simulink model "s_c107m32k_vlbi"  (R2018a)
settings: Solver=VariableStepDiscrete  StartTime=0.0  StopTime=(2^15)*10  RelTol=1e-3
undefined symbols (not defined in the file): fft_stages, n_bits_xengs
libraries: xbsIndex_r4 x23049, casper_library_misc x45, xps_library x4, casper_library_scopes x3, simulink x2
(part 96 of 201)

== system s_c107m32k_vlbi/cd_hmc/hmc_delay/ctrl_pol1 ==
  note: Stall the address increment by 1 cycle as two
      | 128bit words need to be concatenated into one 256bit word
  note: Add a 512 address offset. This is so that the read and write dont clash,
      | and to allow sufficicient time for the HMC to perform the write transactione
      | BEFORE a read transaction on that same write address.
  note: If a sync arrives on a non-valid cycle (should never happen!),
      | latch it and insert it with the first next valid word.
  hmc_sel : Inport
  sync_in : Inport  Port=2
  data_in : Inport  Port=3
  valid_in : Inport  Port=4
  delay_setpoint : Inport  Port=5
  hmc_rdy : Inport  Port=6
  AddSub : xbsIndex_r4/AddSub  mode=Subtraction  use_carryin=off  use_carryout=off  en=off  latency=1  precision=User Defined  arith_type=Unsigned  n_bits=n_bits_max_delay+1  bin_pt=0  quantization=Truncate  overflow=Wrap  use_behavioral_HDL=on  hw_selection=Fabric  pipelined=off  use_rpm=on  dbl_ovrd=off  block_type=addsub
  AddSub2 : xbsIndex_r4/AddSub  mode=Addition  use_carryin=off  use_carryout=off  en=off  latency=1  precision=User Defined  arith_type=Unsigned  n_bits=n_bits_max_delay+1  bin_pt=0  quantization=Truncate  overflow=Wrap  use_behavioral_HDL=on  hw_selection=Fabric  pipelined=off  use_rpm=on  dbl_ovrd=off  block_type=addsub
  Concat : xbsIndex_r4/Concat  num_inputs=6  dbl_ovrd=off  block_type=concat
  Concat1 : xbsIndex_r4/Concat  num_inputs=2  dbl_ovrd=off  block_type=concat
  Concat2 : xbsIndex_r4/Concat  num_inputs=2  dbl_ovrd=off  block_type=concat
  Constant : xbsIndex_r4/Constant  const=512  gui_display_data_type=Fixed-point  arith_type=Unsigned  n_bits=10  bin_pt=0  preci_type=Single  exp_width=8  frac_width=24  explicit_period=on  period=1  equ=P=C  opselect=C  inp2=PCIN>>17  opr=+  inp1=P  carry=CIN  dbl_ovrd=off  block_type=constant
  Constant1 : xbsIndex_r4/Constant  const=0  gui_display_data_type=Fixed-point  arith_type=Unsigned  n_bits=1  bin_pt=0  preci_type=Single  exp_width=8  frac_width=24  explicit_period=on  period=1  equ=P=C  opselect=C  inp2=PCIN>>17  opr=+  inp1=P  carry=CIN  dbl_ovrd=off  block_type=constant
  Constant2 : xbsIndex_r4/Constant  const=1  gui_display_data_type=Fixed-point  arith_type=Unsigned  n_bits=1  bin_pt=0  preci_type=Single  exp_width=8  frac_width=24  explicit_period=on  period=1  equ=P=C  opselect=C  inp2=PCIN>>17  opr=+  inp1=P  carry=CIN  dbl_ovrd=off  block_type=constant
  Constant7 : xbsIndex_r4/Constant  const=1  gui_display_data_type=Fixed-point  arith_type=Unsigned  n_bits=1  bin_pt=0  preci_type=Single  exp_width=8  frac_width=24  explicit_period=on  period=1  equ=P=C  opselect=C  inp2=PCIN>>17  opr=+  inp1=P  carry=CIN  dbl_ovrd=off  block_type=constant
  Convert1 : xbsIndex_r4/Convert  gui_display_data_type=Boolean  arith_type=Boolean  n_bits=16  bin_pt=14  float_type=Single  exp_bits=8  fraction_bits=24  quantization=Truncate  overflow=Wrap  en=off  latency=0  pipeline=off  dbl_ovrd=off  block_type=convert
  Convert6 : xbsIndex_r4/Convert  gui_display_data_type=Fixed-point  arith_type=Unsigned  n_bits=1  bin_pt=0  float_type=Single  exp_bits=8  fraction_bits=24  quantization=Truncate  overflow=Wrap  en=off  latency=0  pipeline=off  dbl_ovrd=off  block_type=convert
  Counter1 : xbsIndex_r4/Counter  cnt_type=Free Running  cnt_to=1  operation=Up  start_count=0  cnt_by_val=1  arith_type=Unsigned  n_bits=9  bin_pt=0  load_pin=off  rst=on  en=on  explicit_period=on  period=1  use_behavioral_HDL=off  implementation=Fabric  dbl_ovrd=off  block_type=counter
  Delay{1..3,5..6,9,11..12,22,28} (10 alike) : xbsIndex_r4/Delay  rst=off  infoeditControl=Selection of Reset will increase slice count due to use of real FFs and instead of SRLs  en=off  latency=2  reg_retiming=on  dbl_ovrd=off  block_type=delay
      settings: block_version=11.4
  Delay{4,10,16,20..21,23..24,31,35..36} (10 alike) : xbsIndex_r4/Delay  rst=off  infoeditControl=Selection of Reset will increase slice count due to use of real FFs and instead of SRLs  en=off  latency=1  reg_retiming=on  dbl_ovrd=off  block_type=delay
      settings: block_version=11.4
  Gateway Out{,1..11} (12 alike) : xbsIndex_r4/Gateway Out  inherit_from_input=off  hdl_port=on  rows=1  columns=1  UseAsDAC=off  DACChannel='1'  interface=None  automatic_assignment=on  address_offset=hex2dec('00')  intf_name=''  intf_description=''  timing_constraint=None  locs_specified=off  LOCs={}  io_standard={}  block_type=gatewayout
  Inverter : xbsIndex_r4/Inverter  en=off  latency=0  dbl_ovrd=off  block_type=inv
  Logical1 : xbsIndex_r4/Logical  logical_function=AND  inputs=2  en=off  latency=0  precision=Full  arith_type=Unsigned  n_bits=16  bin_pt=0  align_bp=on  dbl_ovrd=off  block_type=logical
  Logical27 : xbsIndex_r4/Logical  logical_function=AND  inputs=2  en=off  latency=0  precision=Full  arith_type=Unsigned  n_bits=16  bin_pt=0  align_bp=on  dbl_ovrd=off  block_type=logical
  Register : xbsIndex_r4/Register  init=0  rst=on  en=on  dbl_ovrd=off  block_type=register
  Register1 : xbsIndex_r4/Register  init=0  rst=off  en=on  dbl_ovrd=off  block_type=register
  Slice1 : xbsIndex_r4/Slice  nbits=32  boolean_output=off  mode=Lower Bit Location + Width  bit1=0  base1=MSB of Input  bit0=0  base0=LSB of Input  dbl_ovrd=off  block_type=slice
  Slice2 : xbsIndex_r4/Slice  nbits=32  boolean_output=off  mode=Lower Bit Location + Width  bit1=0  base1=MSB of Input  bit0=0  base0=LSB of Input  dbl_ovrd=off  block_type=slice
  add_parity : Subsystem
  addr : xbsIndex_r4/Counter  cnt_type=Free Running  cnt_to=Inf  operation=Up  start_count=0  cnt_by_val=1  arith_type=Unsigned  n_bits=n_bits_max_delay+1  bin_pt=0  load_pin=off  rst=on  en=on  explicit_period=on  period=1  use_behavioral_HDL=on  implementation=DSP48  use_rpm=off  dbl_ovrd=off  block_type=counter
  addr_stall : xbsIndex_r4/Counter  cnt_type=Count Limited  cnt_to=1  operation=Up  start_count=0  cnt_by_val=1  arith_type=Unsigned  n_bits=1  bin_pt=0  load_pin=off  rst=on  en=on  explicit_period=on  period=1  use_behavioral_HDL=on  implementation=DSP48  use_rpm=off  dbl_ovrd=off  block_type=counter
  innards : Scope  NumInputPorts=4
  innards1 : Scope  NumInputPorts=4
  wait_logic : Scope  NumInputPorts=4
  hmc_wraddr : Outport
  hmc_win : Outport  Port=2
  hmc_rin : Outport  Port=3
  hmc_raddr : Outport  Port=4
  hmc_din_256 : Outport  Port=5
  hmc_tag : Outport  Port=6
  wires:
  Gateway Out8/1 -> wait_logic/1
  Gateway Out9/1 -> wait_logic/2
  Gateway Out10/1 -> wait_logic/3
  Gateway Out11/1 -> wait_logic/4
  Slice2/1 -> Gateway Out3/1
  delay_setpoint/1 -> AddSub2/2
  Constant/1 -> AddSub2/1
  Gateway Out7/1 -> innards1/4
  Gateway Out6/1 -> innards1/3
  Gateway Out5/1 -> innards1/2
  Gateway Out2/1 -> innards1/1
  Slice1/1 -> Gateway Out4/1
  Gateway Out4/1 -> innards/4
  Gateway Out3/1 -> innards/3
  Gateway Out1/1 -> innards/2
  Gateway Out/1 -> innards/1
  Inverter/1 -> Convert6/1
  Convert6/1 -> Concat/5
  Register/1 -> Inverter/1, Gateway Out7/1
  Delay23/1 -> Delay4/1
  Delay21/1 -> Delay10/1
  Delay20/1 -> Delay36/1
  Delay16/1 -> Delay31/1
  Delay5/1 -> Counter1/2, hmc_rin/1, hmc_win/1, Gateway Out1/1, Gateway Out5/1, Register/1, Register/3
  Delay12/1 -> Gateway Out6/1, Register/2, Counter1/1
  Concat2/1 -> hmc_raddr/1
  Concat1/1 -> hmc_wraddr/1, Gateway Out/1, Gateway Out2/1
  Delay1/1 -> Register1/2
  Delay4/1 -> Delay2/1
  Delay2/1 -> Delay1/1
  Delay10/1 -> add_parity/1(din)
  Constant1/1 -> Concat/2
  Constant7/1 -> Concat/4
  Concat/1 -> hmc_din_256/1
  Constant2/1 -> Concat/1
  Logical1/1 -> Delay16/1, addr/2, Gateway Out11/1
  sync_in/1 -> addr_stall/1, Gateway Out8/1, addr/1, Delay20/1
  valid_in/1 -> Logical27/1, Gateway Out9/1, Delay23/1, Logical1/1
  hmc_rdy/1 -> Logical27/2
  Convert1/1 -> Logical1/2
  AddSub2/1 -> AddSub/2
  Logical27/1 -> addr_stall/2
  AddSub/1 -> Delay22/1  "rd_add_HR"
  addr_stall/1 -> Convert1/1, Gateway Out10/1  "stall"
  addr/1 -> Delay35/1  "addr"
  data_in/1 -> Delay21/1  "d_in"
  Delay35/1 -> Delay24/1, AddSub/1
  hmc_sel/1 -> Concat1/2, Concat2/2
  Delay6/1 -> Concat1/1
  Delay11/1 -> Concat2/1
  Delay9/1 -> Delay6/1
  Delay36/1 -> Delay3/1
  Delay31/1 -> Delay28/1
  Delay3/1 -> Delay12/1
  Delay22/1 -> Delay11/1
  Delay28/1 -> Delay5/1
  Register1/1 -> Concat/6, Slice1/1
  Counter1/1 -> hmc_tag/1
  Delay24/1 -> Delay9/1
  add_parity/1(dout) -> Register1/1, Slice2/1, Concat/3  "reg_din"

== system s_c107m32k_vlbi/cd_hmc/hmc_delay/parity_check0 ==
  en : Inport
  din : Inport  Port=2
  Delay1 : xbsIndex_r4/Delay  rst=off  infoeditControl=Selection of Reset will increase slice count due to use of real FFs and instead of SRLs  en=off  latency=3  reg_retiming=on  dbl_ovrd=off  block_type=delay
  Delay2 : xbsIndex_r4/Delay  rst=off  infoeditControl=Selection of Reset will increase slice count due to use of real FFs and instead of SRLs  en=off  latency=2  reg_retiming=on  dbl_ovrd=off  block_type=delay
  Slice : xbsIndex_r4/Slice  nbits=80  boolean_output=off  mode=Lower Bit Location + Width  bit1=0  base1=MSB of Input  bit0=0  base0=LSB of Input  dbl_ovrd=off  block_type=slice
  Slice1 : xbsIndex_r4/Slice  nbits=1  boolean_output=on  mode=Upper Bit Location + Width  bit1=0  base1=MSB of Input  bit0=0  base0=LSB of Input  dbl_ovrd=off  block_type=slice
  bus_expand : Subsystem  mask(bus_expand){mode=divisions of equal size, outputNum=81, outputWidth=1, outputBinaryPt=0, outputArithmeticType=0, show_format=off, outputToWorkspace=off, variablePrefix=out, outputToModelAsWell=on}
      mask prompts: outputNum "Number of outputs:"; outputWidth "Output width:"; outputBinaryPt "Output binary point position:"; outputArithmeticType "Output arithmetic type (ufix=0, fix=1, bool=2):"; show_format "Print format string?"; outputToWorkspace "Output to workspace?"; variablePrefix "Variable name prefix:"; outputToModelAsWell "Output to model as well?"
      mask help:
      | Expands a 'bus' made using a bus_create or Xilinx
      | concat block.
      | The input will be divided into the specified number
      | of outputs with the specified arithmetic types.
      | Divisions are made from most significant bit.
      mask init: same as s_c107m32k_vlbi/bus_expand1
      settings: AttributesFormatString=81 outputs
      mask TypeOptions mode: divisions of equal size | divisions of arbitrary size
      mask Callback mode: bus_expand_callback();
      mask Callback outputWidth: bus_expand_callback();
      mask Callback outputToWorkspace: bus_expand_callback();
  parity : xbsIndex_r4/Logical  logical_function=XOR  inputs=81  en=off  latency=2  precision=User Defined  arith_type=Boolean  n_bits=1  bin_pt=0  align_bp=on  dbl_ovrd=off  block_type=logical
  parity_error : xbsIndex_r4/Logical  logical_function=AND  inputs=2  en=off  latency=1  precision=User Defined  arith_type=Boolean  n_bits=1  bin_pt=0  align_bp=on  dbl_ovrd=off  block_type=logical
  dout : Outport
  error : Outport  Port=2
  wires:
  bus_expand/25(out57) -> parity/25
  bus_expand/29(out53) -> parity/29
  bus_expand/35(out47) -> parity/35
  bus_expand/32(out50) -> parity/32
  bus_expand/23(out59) -> parity/23
  bus_expand/26(out56) -> parity/26
  bus_expand/52(out30) -> parity/52
  bus_expand/30(out52) -> parity/30
  bus_expand/63(out19) -> parity/63
  bus_expand/57(out25) -> parity/57
  bus_expand/17(out65) -> parity/17
  bus_expand/50(out32) -> parity/50
  bus_expand/42(out40) -> parity/42
  bus_expand/19(out63) -> parity/19
  bus_expand/9(out73) -> parity/9
  bus_expand/15(out67) -> parity/15
  bus_expand/16(out66) -> parity/16
  bus_expand/3(out79) -> parity/3
  bus_expand/34(out48) -> parity/34
  bus_expand/37(out45) -> parity/37
  bus_expand/59(out23) -> parity/59
  bus_expand/45(out37) -> parity/45
  bus_expand/48(out34) -> parity/48
  bus_expand/69(out13) -> parity/69
  bus_expand/10(out72) -> parity/10
  bus_expand/47(out35) -> parity/47
  bus_expand/2(out80) -> parity/2
  bus_expand/55(out27) -> parity/55
  bus_expand/6(out76) -> parity/6
  bus_expand/39(out43) -> parity/39
  bus_expand/60(out22) -> parity/60
  bus_expand/65(out17) -> parity/65
  bus_expand/28(out54) -> parity/28
  bus_expand/12(out70) -> parity/12
  bus_expand/66(out16) -> parity/66
  bus_expand/75(out7) -> parity/75
  bus_expand/80(out2) -> parity/80
  bus_expand/36(out46) -> parity/36
  bus_expand/67(out15) -> parity/67
  bus_expand/4(out78) -> parity/4
  bus_expand/41(out41) -> parity/41
  bus_expand/49(out33) -> parity/49
  bus_expand/1(msb_out81) -> parity/1
  bus_expand/71(out11) -> parity/71
  bus_expand/7(out75) -> parity/7
  bus_expand/68(out14) -> parity/68
  bus_expand/33(out49) -> parity/33
  bus_expand/53(out29) -> parity/53
  bus_expand/13(out69) -> parity/13
  bus_expand/5(out77) -> parity/5
  bus_expand/73(out9) -> parity/73
  bus_expand/81(lsb_out1) -> parity/81
  bus_expand/74(out8) -> parity/74
  bus_expand/18(out64) -> parity/18
  bus_expand/14(out68) -> parity/14
  bus_expand/61(out21) -> parity/61
  bus_expand/70(out12) -> parity/70
  bus_expand/64(out18) -> parity/64
  bus_expand/22(out60) -> parity/22
  bus_expand/54(out28) -> parity/54
  bus_expand/20(out62) -> parity/20
  bus_expand/51(out31) -> parity/51
  bus_expand/21(out61) -> parity/21
  bus_expand/40(out42) -> parity/40
  bus_expand/62(out20) -> parity/62
  bus_expand/76(out6) -> parity/76
  bus_expand/38(out44) -> parity/38
  bus_expand/56(out26) -> parity/56
  bus_expand/46(out36) -> parity/46
  bus_expand/72(out10) -> parity/72
  bus_expand/31(out51) -> parity/31
  bus_expand/11(out71) -> parity/11
  bus_expand/77(out5) -> parity/77
  bus_expand/27(out55) -> parity/27
  bus_expand/58(out24) -> parity/58
  bus_expand/44(out38) -> parity/44
  bus_expand/8(out74) -> parity/8
  bus_expand/79(out3) -> parity/79
  bus_expand/24(out58) -> parity/24
  bus_expand/78(out4) -> parity/78
  bus_expand/43(out39) -> parity/43
  Slice1/1 -> parity_error/2
  Delay2/1 -> Slice1/1
  din/1 -> Delay1/1, bus_expand/1(bus_in)
  en/1 -> Delay2/1
  Delay1/1 -> Slice/1
  parity/1 -> parity_error/1
  parity_error/1 -> error/1
  Slice/1 -> dout/1

== system s_c107m32k_vlbi/cd_hmc/hmc_delay/parity_check1 ==
  en : Inport
  din : Inport  Port=2
  Delay1 : xbsIndex_r4/Delay  rst=off  infoeditControl=Selection of Reset will increase slice count due to use of real FFs and instead of SRLs  en=off  latency=3  reg_retiming=on  dbl_ovrd=off  block_type=delay
  Delay2 : xbsIndex_r4/Delay  rst=off  infoeditControl=Selection of Reset will increase slice count due to use of real FFs and instead of SRLs  en=off  latency=2  reg_retiming=on  dbl_ovrd=off  block_type=delay
  Slice : xbsIndex_r4/Slice  nbits=80  boolean_output=off  mode=Lower Bit Location + Width  bit1=0  base1=MSB of Input  bit0=0  base0=LSB of Input  dbl_ovrd=off  block_type=slice
  Slice1 : xbsIndex_r4/Slice  nbits=1  boolean_output=on  mode=Upper Bit Location + Width  bit1=0  base1=MSB of Input  bit0=0  base0=LSB of Input  dbl_ovrd=off  block_type=slice
  bus_expand : Subsystem  mask(bus_expand){mode=divisions of equal size, outputNum=81, outputWidth=1, outputBinaryPt=0, outputArithmeticType=0, show_format=off, outputToWorkspace=off, variablePrefix=out, outputToModelAsWell=on}
      mask prompts: outputNum "Number of outputs:"; outputWidth "Output width:"; outputBinaryPt "Output binary point position:"; outputArithmeticType "Output arithmetic type (ufix=0, fix=1, bool=2):"; show_format "Print format string?"; outputToWorkspace "Output to workspace?"; variablePrefix "Variable name prefix:"; outputToModelAsWell "Output to model as well?"
      mask help:
      | Expands a 'bus' made using a bus_create or Xilinx
      | concat block.
      | The input will be divided into the specified number
      | of outputs with the specified arithmetic types.
      | Divisions are made from most significant bit.
      mask init: same as s_c107m32k_vlbi/bus_expand1
      settings: AttributesFormatString=81 outputs
      mask TypeOptions mode: divisions of equal size | divisions of arbitrary size
      mask Callback mode: bus_expand_callback();
      mask Callback outputWidth: bus_expand_callback();
      mask Callback outputToWorkspace: bus_expand_callback();
  parity : xbsIndex_r4/Logical  logical_function=XOR  inputs=81  en=off  latency=2  precision=User Defined  arith_type=Boolean  n_bits=1  bin_pt=0  align_bp=on  dbl_ovrd=off  block_type=logical
  parity_error : xbsIndex_r4/Logical  logical_function=AND  inputs=2  en=off  latency=1  precision=User Defined  arith_type=Boolean  n_bits=1  bin_pt=0  align_bp=on  dbl_ovrd=off  block_type=logical
  dout : Outport
  error : Outport  Port=2
  wires:
  Slice/1 -> dout/1
  parity_error/1 -> error/1
  parity/1 -> parity_error/1
  Delay1/1 -> Slice/1
  en/1 -> Delay2/1
  din/1 -> bus_expand/1(bus_in), Delay1/1
  Delay2/1 -> Slice1/1
  Slice1/1 -> parity_error/2
  bus_expand/43(out39) -> parity/43
  bus_expand/78(out4) -> parity/78
  bus_expand/24(out58) -> parity/24
  bus_expand/79(out3) -> parity/79
  bus_expand/8(out74) -> parity/8
  bus_expand/44(out38) -> parity/44
  bus_expand/58(out24) -> parity/58
  bus_expand/27(out55) -> parity/27
  bus_expand/77(out5) -> parity/77
  bus_expand/11(out71) -> parity/11
  bus_expand/31(out51) -> parity/31
  bus_expand/72(out10) -> parity/72
  bus_expand/46(out36) -> parity/46
  bus_expand/56(out26) -> parity/56
  bus_expand/38(out44) -> parity/38
  bus_expand/76(out6) -> parity/76
  bus_expand/62(out20) -> parity/62
  bus_expand/40(out42) -> parity/40
  bus_expand/21(out61) -> parity/21
  bus_expand/51(out31) -> parity/51
  bus_expand/20(out62) -> parity/20
  bus_expand/54(out28) -> parity/54
  bus_expand/22(out60) -> parity/22
  bus_expand/64(out18) -> parity/64
  bus_expand/70(out12) -> parity/70
  bus_expand/61(out21) -> parity/61
  bus_expand/14(out68) -> parity/14
  bus_expand/18(out64) -> parity/18
  bus_expand/74(out8) -> parity/74
  bus_expand/81(lsb_out1) -> parity/81
  bus_expand/73(out9) -> parity/73
  bus_expand/5(out77) -> parity/5
  bus_expand/13(out69) -> parity/13
  bus_expand/53(out29) -> parity/53
  bus_expand/33(out49) -> parity/33
  bus_expand/68(out14) -> parity/68
  bus_expand/7(out75) -> parity/7
  bus_expand/71(out11) -> parity/71
  bus_expand/1(msb_out81) -> parity/1
  bus_expand/49(out33) -> parity/49
  bus_expand/41(out41) -> parity/41
  bus_expand/4(out78) -> parity/4
  bus_expand/67(out15) -> parity/67
  bus_expand/36(out46) -> parity/36
  bus_expand/80(out2) -> parity/80
  bus_expand/75(out7) -> parity/75
  bus_expand/66(out16) -> parity/66
  bus_expand/12(out70) -> parity/12
  bus_expand/28(out54) -> parity/28
  bus_expand/65(out17) -> parity/65
  bus_expand/60(out22) -> parity/60
  bus_expand/39(out43) -> parity/39
  bus_expand/6(out76) -> parity/6
  bus_expand/55(out27) -> parity/55
  bus_expand/2(out80) -> parity/2
  bus_expand/47(out35) -> parity/47
  bus_expand/10(out72) -> parity/10
  bus_expand/69(out13) -> parity/69
  bus_expand/48(out34) -> parity/48
  bus_expand/45(out37) -> parity/45
  bus_expand/59(out23) -> parity/59
  bus_expand/37(out45) -> parity/37
  bus_expand/34(out48) -> parity/34
  bus_expand/3(out79) -> parity/3
  bus_expand/16(out66) -> parity/16
  bus_expand/15(out67) -> parity/15
  bus_expand/9(out73) -> parity/9
  bus_expand/19(out63) -> parity/19
  bus_expand/42(out40) -> parity/42
  bus_expand/50(out32) -> parity/50
  bus_expand/17(out65) -> parity/17
  bus_expand/57(out25) -> parity/57
  bus_expand/63(out19) -> parity/63
  bus_expand/30(out52) -> parity/30
  bus_expand/52(out30) -> parity/52
  bus_expand/26(out56) -> parity/26
  bus_expand/23(out59) -> parity/23
  bus_expand/32(out50) -> parity/32
  bus_expand/35(out47) -> parity/35
  bus_expand/29(out53) -> parity/29
  bus_expand/25(out57) -> parity/25

== system s_c107m32k_vlbi/cd_hmc/hmc_delay/pipeline1 ==
  d : Inport
  Register0 : xbsIndex_r4/Register  init=0  rst=off  en=off  dbl_ovrd=off  block_type=register
      settings: block_version=11.4
  Register1 : xbsIndex_r4/Register  init=0  rst=off  en=off  dbl_ovrd=off  block_type=register
      settings: block_version=11.4
  q : Outport
  wires:
  Register1/1 -> q/1
  d/1 -> Register0/1
  Register0/1 -> Register1/1

== system s_c107m32k_vlbi/cd_hmc/hmc_delay/pipeline11 ==
  d : Inport
  Register0 : xbsIndex_r4/Register  init=0  rst=off  en=off  dbl_ovrd=off  block_type=register
      settings: block_version=11.4
  Register1 : xbsIndex_r4/Register  init=0  rst=off  en=off  dbl_ovrd=off  block_type=register
      settings: block_version=11.4
  q : Outport
  wires:
  Register1/1 -> q/1
  d/1 -> Register0/1
  Register0/1 -> Register1/1

== system s_c107m32k_vlbi/cd_hmc/hmc_delay/pipeline115 ==
  d : Inport
  Register0 : xbsIndex_r4/Register  init=0  rst=off  en=off  dbl_ovrd=off  block_type=register
      settings: block_version=11.4
  Register1 : xbsIndex_r4/Register  init=0  rst=off  en=off  dbl_ovrd=off  block_type=register
      settings: block_version=11.4
  q : Outport
  wires:
  Register1/1 -> q/1
  d/1 -> Register0/1
  Register0/1 -> Register1/1

== system s_c107m32k_vlbi/cd_hmc/hmc_delay/pipeline116 ==
  d : Inport
  Register0 : xbsIndex_r4/Register  init=0  rst=off  en=off  dbl_ovrd=off  block_type=register
      settings: block_version=11.4
  Register1 : xbsIndex_r4/Register  init=0  rst=off  en=off  dbl_ovrd=off  block_type=register
      settings: block_version=11.4
  q : Outport
  wires:
  Register1/1 -> q/1
  d/1 -> Register0/1
  Register0/1 -> Register1/1

== system s_c107m32k_vlbi/cd_hmc/hmc_delay/pipeline117 ==
  d : Inport
  Register0 : xbsIndex_r4/Register  init=0  rst=off  en=off  dbl_ovrd=off  block_type=register
      settings: block_version=11.4
  Register1 : xbsIndex_r4/Register  init=0  rst=off  en=off  dbl_ovrd=off  block_type=register
      settings: block_version=11.4
  q : Outport
  wires:
  Register1/1 -> q/1
  d/1 -> Register0/1
  Register0/1 -> Register1/1

== system s_c107m32k_vlbi/cd_hmc/hmc_delay/pipeline12 ==
  d : Inport
  Register0 : xbsIndex_r4/Register  init=0  rst=off  en=off  dbl_ovrd=off  block_type=register
      settings: block_version=11.4
  q : Outport
  wires:
  Register0/1 -> q/1
  d/1 -> Register0/1

== system s_c107m32k_vlbi/cd_hmc/hmc_delay/pipeline13 ==
  d : Inport
  Register0 : xbsIndex_r4/Register  init=0  rst=off  en=off  dbl_ovrd=off  block_type=register
      settings: block_version=11.4
  Register1 : xbsIndex_r4/Register  init=0  rst=off  en=off  dbl_ovrd=off  block_type=register
      settings: block_version=11.4
  q : Outport
  wires:
  Register1/1 -> q/1
  d/1 -> Register0/1
  Register0/1 -> Register1/1

== system s_c107m32k_vlbi/cd_hmc/hmc_delay/pipeline15 ==
  d : Inport
  Register0 : xbsIndex_r4/Register  init=0  rst=off  en=off  dbl_ovrd=off  block_type=register
      settings: block_version=11.4
  Register1 : xbsIndex_r4/Register  init=0  rst=off  en=off  dbl_ovrd=off  block_type=register
      settings: block_version=11.4
  q : Outport
  wires:
  Register1/1 -> q/1
  d/1 -> Register0/1
  Register0/1 -> Register1/1

== system s_c107m32k_vlbi/cd_hmc/hmc_delay/pipeline152 ==
  d : Inport
  Register0 : xbsIndex_r4/Register  init=0  rst=off  en=off  dbl_ovrd=off  block_type=register
      settings: block_version=11.4
  Register1 : xbsIndex_r4/Register  init=0  rst=off  en=off  dbl_ovrd=off  block_type=register
      settings: block_version=11.4
  q : Outport
  wires:
  Register1/1 -> q/1
  d/1 -> Register0/1
  Register0/1 -> Register1/1

== system s_c107m32k_vlbi/cd_hmc/hmc_delay/pipeline153 ==
  d : Inport
  Register0 : xbsIndex_r4/Register  init=0  rst=off  en=off  dbl_ovrd=off  block_type=register
      settings: block_version=11.4
  Register1 : xbsIndex_r4/Register  init=0  rst=off  en=off  dbl_ovrd=off  block_type=register
      settings: block_version=11.4
  q : Outport
  wires:
  Register1/1 -> q/1
  d/1 -> Register0/1
  Register0/1 -> Register1/1

== system s_c107m32k_vlbi/cd_hmc/hmc_delay/pipeline154 ==
  d : Inport
  Register0 : xbsIndex_r4/Register  init=0  rst=off  en=off  dbl_ovrd=off  block_type=register
      settings: block_version=11.4
  Register1 : xbsIndex_r4/Register  init=0  rst=off  en=off  dbl_ovrd=off  block_type=register
      settings: block_version=11.4
  q : Outport
  wires:
  Register1/1 -> q/1
  d/1 -> Register0/1
  Register0/1 -> Register1/1

== system s_c107m32k_vlbi/cd_hmc/hmc_delay/pipeline16 ==
  d : Inport
  Register0 : xbsIndex_r4/Register  init=0  rst=off  en=off  dbl_ovrd=off  block_type=register
      settings: block_version=11.4
  Register1 : xbsIndex_r4/Register  init=0  rst=off  en=off  dbl_ovrd=off  block_type=register
      settings: block_version=11.4
  q : Outport
  wires:
  Register1/1 -> q/1
  d/1 -> Register0/1
  Register0/1 -> Register1/1

== system s_c107m32k_vlbi/cd_hmc/hmc_delay/pipeline168 ==
  d : Inport
  Register0 : xbsIndex_r4/Register  init=0  rst=off  en=off  dbl_ovrd=off  block_type=register
      settings: block_version=11.4
  Register1 : xbsIndex_r4/Register  init=0  rst=off  en=off  dbl_ovrd=off  block_type=register
      settings: block_version=11.4
  q : Outport
  wires:
  Register1/1 -> q/1
  d/1 -> Register0/1
  Register0/1 -> Register1/1

== system s_c107m32k_vlbi/cd_hmc/hmc_delay/pipeline169 ==
  d : Inport
  Register0 : xbsIndex_r4/Register  init=0  rst=off  en=off  dbl_ovrd=off  block_type=register
      settings: block_version=11.4
  Register1 : xbsIndex_r4/Register  init=0  rst=off  en=off  dbl_ovrd=off  block_type=register
      settings: block_version=11.4
  q : Outport
  wires:
  Register1/1 -> q/1
  d/1 -> Register0/1
  Register0/1 -> Register1/1

== system s_c107m32k_vlbi/cd_hmc/hmc_delay/pipeline171 ==
  d : Inport
  Register0 : xbsIndex_r4/Register  init=0  rst=off  en=off  dbl_ovrd=off  block_type=register
      settings: block_version=11.4
  Register1 : xbsIndex_r4/Register  init=0  rst=off  en=off  dbl_ovrd=off  block_type=register
      settings: block_version=11.4
  q : Outport
  wires:
  Register1/1 -> q/1
  d/1 -> Register0/1
  Register0/1 -> Register1/1

== system s_c107m32k_vlbi/cd_hmc/hmc_delay/pipeline172 ==
  d : Inport
  Register0 : xbsIndex_r4/Register  init=0  rst=off  en=off  dbl_ovrd=off  block_type=register
      settings: block_version=11.4
  Register1 : xbsIndex_r4/Register  init=0  rst=off  en=off  dbl_ovrd=off  block_type=register
      settings: block_version=11.4
  q : Outport
  wires:
  Register1/1 -> q/1
  d/1 -> Register0/1
  Register0/1 -> Register1/1

== system s_c107m32k_vlbi/cd_hmc/hmc_delay/pipeline174 ==
  d : Inport
  Register0 : xbsIndex_r4/Register  init=0  rst=off  en=off  dbl_ovrd=off  block_type=register
      settings: block_version=11.4
  Register1 : xbsIndex_r4/Register  init=0  rst=off  en=off  dbl_ovrd=off  block_type=register
      settings: block_version=11.4
  q : Outport
  wires:
  Register1/1 -> q/1
  d/1 -> Register0/1
  Register0/1 -> Register1/1

== system s_c107m32k_vlbi/cd_hmc/hmc_delay/pipeline18 ==
  d : Inport
  Register0 : xbsIndex_r4/Register  init=0  rst=off  en=off  dbl_ovrd=off  block_type=register
      settings: block_version=11.4
  q : Outport
  wires:
  Register0/1 -> q/1
  d/1 -> Register0/1

== system s_c107m32k_vlbi/cd_hmc/hmc_delay/pipeline19 ==
  d : Inport
  Register0 : xbsIndex_r4/Register  init=0  rst=off  en=off  dbl_ovrd=off  block_type=register
      settings: block_version=11.4
  Register1 : xbsIndex_r4/Register  init=0  rst=off  en=off  dbl_ovrd=off  block_type=register
      settings: block_version=11.4
  q : Outport
  wires:
  Register1/1 -> q/1
  d/1 -> Register0/1
  Register0/1 -> Register1/1

== system s_c107m32k_vlbi/cd_hmc/hmc_delay/pipeline2 ==
  d : Inport
  Register0 : xbsIndex_r4/Register  init=0  rst=off  en=off  dbl_ovrd=off  block_type=register
      settings: block_version=11.4
  Register1 : xbsIndex_r4/Register  init=0  rst=off  en=off  dbl_ovrd=off  block_type=register
      settings: block_version=11.4
  q : Outport
  wires:
  Register1/1 -> q/1
  d/1 -> Register0/1
  Register0/1 -> Register1/1

== system s_c107m32k_vlbi/cd_hmc/hmc_delay/pipeline20 ==
  d : Inport
  Register0 : xbsIndex_r4/Register  init=0  rst=off  en=off  dbl_ovrd=off  block_type=register
      settings: block_version=11.4
  Register1 : xbsIndex_r4/Register  init=0  rst=off  en=off  dbl_ovrd=off  block_type=register
      settings: block_version=11.4
  q : Outport
  wires:
  Register1/1 -> q/1
  d/1 -> Register0/1
  Register0/1 -> Register1/1

== system s_c107m32k_vlbi/cd_hmc/hmc_delay/pipeline21 ==
  d : Inport
  Register0 : xbsIndex_r4/Register  init=0  rst=off  en=off  dbl_ovrd=off  block_type=register
      settings: block_version=11.4
  Register1 : xbsIndex_r4/Register  init=0  rst=off  en=off  dbl_ovrd=off  block_type=register
      settings: block_version=11.4
  q : Outport
  wires:
  Register1/1 -> q/1
  d/1 -> Register0/1
  Register0/1 -> Register1/1

== system s_c107m32k_vlbi/cd_hmc/hmc_delay/pipeline22 ==
  d : Inport
  Register0 : xbsIndex_r4/Register  init=0  rst=off  en=off  dbl_ovrd=off  block_type=register
      settings: block_version=11.4
  Register1 : xbsIndex_r4/Register  init=0  rst=off  en=off  dbl_ovrd=off  block_type=register
      settings: block_version=11.4
  q : Outport
  wires:
  Register1/1 -> q/1
  d/1 -> Register0/1
  Register0/1 -> Register1/1

== system s_c107m32k_vlbi/cd_hmc/hmc_delay/pipeline23 ==
  d : Inport
  Register0 : xbsIndex_r4/Register  init=0  rst=off  en=off  dbl_ovrd=off  block_type=register
      settings: block_version=11.4
  Register1 : xbsIndex_r4/Register  init=0  rst=off  en=off  dbl_ovrd=off  block_type=register
      settings: block_version=11.4
  q : Outport
  wires:
  Register1/1 -> q/1
  d/1 -> Register0/1
  Register0/1 -> Register1/1

== system s_c107m32k_vlbi/cd_hmc/hmc_delay/pipeline24 ==
  d : Inport
  Register0 : xbsIndex_r4/Register  init=0  rst=off  en=off  dbl_ovrd=off  block_type=register
      settings: block_version=11.4
  Register1 : xbsIndex_r4/Register  init=0  rst=off  en=off  dbl_ovrd=off  block_type=register
      settings: block_version=11.4
  q : Outport
  wires:
  Register1/1 -> q/1
  d/1 -> Register0/1
  Register0/1 -> Register1/1

== system s_c107m32k_vlbi/cd_hmc/hmc_delay/pipeline26 ==
  d : Inport
  Register0 : xbsIndex_r4/Register  init=0  rst=off  en=off  dbl_ovrd=off  block_type=register
      settings: block_version=11.4
  Register1 : xbsIndex_r4/Register  init=0  rst=off  en=off  dbl_ovrd=off  block_type=register
      settings: block_version=11.4
  q : Outport
  wires:
  Register1/1 -> q/1
  d/1 -> Register0/1
  Register0/1 -> Register1/1

== system s_c107m32k_vlbi/cd_hmc/hmc_delay/pipeline27 ==
  d : Inport
  Register0 : xbsIndex_r4/Register  init=0  rst=off  en=off  dbl_ovrd=off  block_type=register
      settings: block_version=11.4
  Register1 : xbsIndex_r4/Register  init=0  rst=off  en=off  dbl_ovrd=off  block_type=register
      settings: block_version=11.4
  q : Outport
  wires:
  Register1/1 -> q/1
  d/1 -> Register0/1
  Register0/1 -> Register1/1

== system s_c107m32k_vlbi/cd_hmc/hmc_delay/pipeline3 ==
  d : Inport
  Register0 : xbsIndex_r4/Register  init=0  rst=off  en=off  dbl_ovrd=off  block_type=register
      settings: block_version=11.4
  Register1 : xbsIndex_r4/Register  init=0  rst=off  en=off  dbl_ovrd=off  block_type=register
      settings: block_version=11.4
  q : Outport
  wires:
  Register1/1 -> q/1
  d/1 -> Register0/1
  Register0/1 -> Register1/1

== system s_c107m32k_vlbi/cd_hmc/hmc_delay/pipeline5 ==
  d : Inport
  Register0 : xbsIndex_r4/Register  init=0  rst=off  en=off  dbl_ovrd=off  block_type=register
      settings: block_version=11.4
  Register1 : xbsIndex_r4/Register  init=0  rst=off  en=off  dbl_ovrd=off  block_type=register
      settings: block_version=11.4
  q : Outport
  wires:
  Register1/1 -> q/1
  d/1 -> Register0/1
  Register0/1 -> Register1/1

== system s_c107m32k_vlbi/cd_hmc/hmc_delay/pipeline61 ==
  d : Inport
  Register0 : xbsIndex_r4/Register  init=0  rst=off  en=off  dbl_ovrd=off  block_type=register
      settings: block_version=11.4
  Register1 : xbsIndex_r4/Register  init=0  rst=off  en=off  dbl_ovrd=off  block_type=register
      settings: block_version=11.4
  q : Outport
  wires:
  Register1/1 -> q/1
  d/1 -> Register0/1
  Register0/1 -> Register1/1

== system s_c107m32k_vlbi/cd_hmc/hmc_delay/pipeline79 ==
  d : Inport
  Register0 : xbsIndex_r4/Register  init=0  rst=off  en=off  dbl_ovrd=off  block_type=register
      settings: block_version=11.4
  Register1 : xbsIndex_r4/Register  init=0  rst=off  en=off  dbl_ovrd=off  block_type=register
      settings: block_version=11.4
  q : Outport
  wires:
  Register1/1 -> q/1
  d/1 -> Register0/1
  Register0/1 -> Register1/1

== system s_c107m32k_vlbi/cd_hmc/hmc_delay/pipeline8 ==
  d : Inport
  Register0 : xbsIndex_r4/Register  init=0  rst=off  en=off  dbl_ovrd=off  block_type=register
      settings: block_version=11.4
  Register1 : xbsIndex_r4/Register  init=0  rst=off  en=off  dbl_ovrd=off  block_type=register
      settings: block_version=11.4
  q : Outport
  wires:
  Register1/1 -> q/1
  d/1 -> Register0/1
  Register0/1 -> Register1/1

== system s_c107m32k_vlbi/cd_hmc/hmc_delay/pipeline9 ==
  d : Inport
  Register0 : xbsIndex_r4/Register  init=0  rst=off  en=off  dbl_ovrd=off  block_type=register
      settings: block_version=11.4
  Register1 : xbsIndex_r4/Register  init=0  rst=off  en=off  dbl_ovrd=off  block_type=register
      settings: block_version=11.4
  q : Outport
  wires:
  Register1/1 -> q/1
  d/1 -> Register0/1
  Register0/1 -> Register1/1

== system s_c107m32k_vlbi/cd_hmc/hmc_delay/reord ==
  note: if rd_addr ever gets close to wr_addr, issue slip error
  sync_pol0 : Inport
  tag_in0 : Inport  Port=2
  data_in0 : Inport  Port=3
  valid_in0 : Inport  Port=4
  sync_pol1 : Inport  Port=5
  valid_in1 : Inport  Port=6
  tag_in1 : Inport  Port=7
  data_in1 : Inport  Port=8
  AddSub : xbsIndex_r4/AddSub  mode=Subtraction  use_carryin=off  use_carryout=off  en=off  latency=1  precision=User Defined  arith_type=Unsigned  n_bits=9  bin_pt=0  quantization=Truncate  overflow=Wrap  use_behavioral_HDL=on  hw_selection=Fabric  pipelined=off  dbl_ovrd=off  block_type=addsub
  AddSub1 : xbsIndex_r4/AddSub  mode=Subtraction  use_carryin=off  use_carryout=off  en=off  latency=1  precision=User Defined  arith_type=Unsigned  n_bits=9  bin_pt=0  quantization=Truncate  overflow=Wrap  use_behavioral_HDL=on  hw_selection=Fabric  pipelined=off  dbl_ovrd=off  block_type=addsub
  Constant1 : xbsIndex_r4/Constant  const=32  gui_display_data_type=Fixed-point  arith_type=Unsigned  n_bits=9  bin_pt=0  preci_type=Single  exp_width=8  frac_width=24  explicit_period=on  period=1  equ=P=C  opselect=C  inp2=PCIN>>17  opr=+  inp1=P  carry=CIN  dbl_ovrd=off  block_type=constant
  Constant2 : xbsIndex_r4/Constant  const=0  gui_display_data_type=Fixed-point  arith_type=Unsigned  n_bits=83  bin_pt=0  preci_type=Single  exp_width=8  frac_width=24  explicit_period=on  period=1  equ=P=C  opselect=C  inp2=PCIN>>17  opr=+  inp1=P  carry=CIN  dbl_ovrd=off  block_type=constant
  Constant3 : xbsIndex_r4/Constant  const=0  gui_display_data_type=Fixed-point  arith_type=Unsigned  n_bits=83  bin_pt=0  preci_type=Single  exp_width=8  frac_width=24  explicit_period=on  period=1  equ=P=C  opselect=C  inp2=PCIN>>17  opr=+  inp1=P  carry=CIN  dbl_ovrd=off  block_type=constant
  Constant4 : xbsIndex_r4/Constant  const=32  gui_display_data_type=Fixed-point  arith_type=Unsigned  n_bits=9  bin_pt=0  preci_type=Single  exp_width=8  frac_width=24  explicit_period=on  period=1  equ=P=C  opselect=C  inp2=PCIN>>17  opr=+  inp1=P  carry=CIN  dbl_ovrd=off  block_type=constant
  Delay{3,5,7,32..34} (6 alike) : xbsIndex_r4/Delay  rst=off  infoeditControl=Selection of Reset will increase slice count due to use of real FFs and instead of SRLs  en=off  latency=1  reg_retiming=on  dbl_ovrd=off  block_type=delay
      settings: infoedit=Hardware notes: A delay line is a chain, each link of which is an SRL16 or SRL32 followed by a flip-flop.  block_version=11.4
  Delay9 : xbsIndex_r4/Delay  rst=off  infoeditControl=Selection of Reset will increase slice count due to use of real FFs and instead of SRLs  en=off  latency=3  reg_retiming=on  dbl_ovrd=off  block_type=delay
      settings: infoedit=Hardware notes: A delay line is a chain, each link of which is an SRL16 or SRL32 followed by a flip-flop.  block_version=11.4
  Logical1 : xbsIndex_r4/Logical  logical_function=AND  inputs=2  en=off  latency=1  precision=Full  arith_type=Unsigned  n_bits=16  bin_pt=0  align_bp=on  dbl_ovrd=off  block_type=logical
  Logical2 : xbsIndex_r4/Logical  logical_function=AND  inputs=2  en=off  latency=1  precision=Full  arith_type=Unsigned  n_bits=16  bin_pt=0  align_bp=on  dbl_ovrd=off  block_type=logical
  Relational : xbsIndex_r4/Relational  mode=a>b  op_type=Bool  en=off  latency=2  dbl_ovrd=off  block_type=relational
  Relational1 : xbsIndex_r4/Relational  mode=a>b  op_type=Bool  en=off  latency=2  dbl_ovrd=off  block_type=relational
  Slice10 : xbsIndex_r4/Slice  nbits=166  boolean_output=off  mode=Lower Bit Location + Width  bit1=0  base1=MSB of Input  bit0=0  base0=LSB of Input  dbl_ovrd=off  block_type=slice
  Slice2 : xbsIndex_r4/Slice  nbits=9  boolean_output=off  mode=Upper Bit Location + Width  bit1=0  base1=MSB of Input  bit0=0  base0=LSB of Input  dbl_ovrd=off  block_type=slice
  Slice6 : xbsIndex_r4/Slice  nbits=166  boolean_output=off  mode=Lower Bit Location + Width  bit1=0  base1=MSB of Input  bit0=0  base0=LSB of Input  dbl_ovrd=off  block_type=slice
  Slice7 : xbsIndex_r4/Slice  nbits=9  boolean_output=off  mode=Upper Bit Location + Width  bit1=0  base1=MSB of Input  bit0=0  base0=LSB of Input  dbl_ovrd=off  block_type=slice
  Terminator1 : Terminator
  Terminator35 : Terminator
  ctrl : Subsystem
  reord_bram : xbsIndex_r4/Dual Port RAM  depth=1024  initVector=zeros(1,1024)  distributed_mem=Block RAM  init_a=0  init_b=0  rst_a=off  rst_b=off  en_a=off  en_b=off  latency=3  write_mode_A=Read Before Write  write_mode_B=Read Before Write  optimize=Speed  dbl_ovrd=off  block_type=dpram
  reord_bram1 : xbsIndex_r4/Dual Port RAM  depth=1024  initVector=zeros(1,1024)  distributed_mem=Block RAM  init_a=0  init_b=0  rst_a=off  rst_b=off  en_a=off  en_b=off  latency=3  write_mode_A=Read Before Write  write_mode_B=Read Before Write  optimize=Speed  dbl_ovrd=off  block_type=dpram
  data_out0 : Outport
  valid_out : Outport  Port=2
  err0 : Outport  Port=3
  data_out1 : Outport  Port=4
  err1 : Outport  Port=5
  wires:
  Relational1/1 -> Logical2/2
  Logical2/1 -> err1/1
  Logical1/1 -> err0/1
  sync_pol0/1 -> ctrl/1(sync_p0)
  Slice7/1 -> AddSub1/1
  Delay32/1 -> AddSub1/2, reord_bram1/4
  AddSub1/1 -> Relational1/2
  Constant4/1 -> Relational1/1
  reord_bram1/1 -> data_out1/1
  Constant3/1 -> reord_bram1/2
  data_in1/1 -> Slice6/1
  tag_in1/1 -> Delay32/1
  Delay33/1 -> reord_bram1/5
  Slice6/1 -> Delay33/1
  Delay34/1 -> reord_bram1/6
  reord_bram1/2 -> Terminator1/1
  valid_in1/1 -> Delay34/1, ctrl/4(dvalid_p1)
  sync_pol1/1 -> ctrl/3(sync_p1)
  reord_bram/1 -> data_out0/1
  Relational/1 -> Logical1/2
  ctrl/2(bram_rd_en) -> reord_bram/3, reord_bram1/3, Delay9/1
  ctrl/1(bram_rd_addr) -> reord_bram/1, Slice2/1, Slice7/1, reord_bram1/1
  Delay3/1 -> reord_bram/4, AddSub/2
  data_in0/1 -> Slice10/1
  tag_in0/1 -> Delay3/1
  valid_in0/1 -> ctrl/2(dvalid_p0), Delay7/1
  Slice2/1 -> AddSub/1
  AddSub/1 -> Relational/2
  Constant1/1 -> Relational/1
  Delay5/1 -> reord_bram/5
  Delay9/1 -> Logical1/1, Logical2/1, valid_out/1
  Slice10/1 -> Delay5/1
  Constant2/1 -> reord_bram/2
  Delay7/1 -> reord_bram/6
  reord_bram/2 -> Terminator35/1

== system s_c107m32k_vlbi/cd_hmc/hmc_delay/snap_in ==
  in_sync0 : Inport
  in_sync1 : Inport  Port=2
  in_data0 : Inport  Port=3
  in_data1 : Inport  Port=4
  in_rd_addr : Inport  Port=5
  in_wr_addr : Inport  Port=6
  in_valid : Inport  Port=7
  in_tag : Inport  Port=8
  we : Inport  Port=9
  trig : Inport  Port=10
  assert_data0 : xbsIndex_r4/Assert  assert_type=on  type_source=Explicitly  gui_display_data_type=Fixed-point  arith_type=Unsigned  n_bits=29  bin_pt=0  preci_type=Single  exp_width=8  frac_width=24  assert_rate=off  rate_source=Explicitly  period=1  output_port=on  block_type=assert
  assert_data1 : xbsIndex_r4/Assert  assert_type=on  type_source=Explicitly  gui_display_data_type=Fixed-point  arith_type=Unsigned  n_bits=29  bin_pt=0  preci_type=Single  exp_width=8  frac_width=24  assert_rate=off  rate_source=Explicitly  period=1  output_port=on  block_type=assert
  assert_rd_addr : xbsIndex_r4/Assert  assert_type=on  type_source=Explicitly  gui_display_data_type=Fixed-point  arith_type=Unsigned  n_bits=29  bin_pt=0  preci_type=Single  exp_width=8  frac_width=24  assert_rate=off  rate_source=Explicitly  period=1  output_port=on  block_type=assert
  assert_sync0 : xbsIndex_r4/Assert  assert_type=on  type_source=Explicitly  gui_display_data_type=Boolean  arith_type=Boolean  n_bits=1  bin_pt=0  preci_type=Single  exp_width=8  frac_width=24  assert_rate=off  rate_source=Explicitly  period=1  output_port=on  block_type=assert
  assert_sync1 : xbsIndex_r4/Assert  assert_type=on  type_source=Explicitly  gui_display_data_type=Boolean  arith_type=Boolean  n_bits=1  bin_pt=0  preci_type=Single  exp_width=8  frac_width=24  assert_rate=off  rate_source=Explicitly  period=1  output_port=on  block_type=assert
  assert_tag : xbsIndex_r4/Assert  assert_type=on  type_source=Explicitly  gui_display_data_type=Fixed-point  arith_type=Unsigned  n_bits=9  bin_pt=0  preci_type=Single  exp_width=8  frac_width=24  assert_rate=off  rate_source=Explicitly  period=1  output_port=on  block_type=assert
  assert_valid : xbsIndex_r4/Assert  assert_type=on  type_source=Explicitly  gui_display_data_type=Boolean  arith_type=Boolean  n_bits=1  bin_pt=0  preci_type=Single  exp_width=8  frac_width=24  assert_rate=off  rate_source=Explicitly  period=1  output_port=on  block_type=assert
  assert_wr_addr : xbsIndex_r4/Assert  assert_type=on  type_source=Explicitly  gui_display_data_type=Fixed-point  arith_type=Unsigned  n_bits=29  bin_pt=0  preci_type=Single  exp_width=8  frac_width=24  assert_rate=off  rate_source=Explicitly  period=1  output_port=on  block_type=assert
  buscreate : Subsystem  AncestorBlock=casper_library_flow_control/bus_create  mask(bus_create){inputNum=8}
      mask prompts: inputNum "Number of inputs:"
      mask init:
      | bus_create_init(gcb,...
      |     'inputNum', inputNum);
  io_delay : Subsystem  AncestorBlock=casper_library_delays/pipeline  mask(pipeline){csp_latency=2}
      mask prompts: csp_latency "Latency"
      mask help:
      | An explicitly laid-out delay line to avoid mapping to SRL16s
      | for use in pipelining to help achieve timing closure.
      mask init:
      | pipeline_init(gcb,'latency',csp_latency);
      settings: AttributesFormatString=Latency = %<latency>
      mask Display:
      | port_label('input', 1, 'd');
      | port_label('output', 1, 'q');
      | disp(['Z^-', num2str(csp_latency)]);
  ss : Subsystem  Tag=casper:snapshot  AncestorBlock=casper_library_scopes/snapshot  mask(snapshot){storage=bram, dram_dimm=2, dram_clock=250, nsamples=9, data_width=128, offset=on, circap=off, value=off, ext_arm=off, ext_circ=off, provide_outputs=off, use_dsp48=on}
      mask prompts: storage "Storage medium"; dram_dimm "DRAM dimm"; dram_clock "DRAM clock rate"; nsamples "Number of Samples (2^?)"; data_width "Data width"; offset "Start delay support"; circap "Circular capture support"; value "Extra value capture support"; ext_arm "External arm support"; ext_circ "External circular capture support"; provide_outputs "Provide outputs"; use_dsp48 "Use DSP48s to implement counters"
      mask help:
      | Standard snap block, but with the following optional extras;
      |  1) Optionally delay the fabric trigger by a user-specified number of valids.
      |  2) Capture continuously after a trigger until a stop pulse is received. Data is captured into BRAM continuously, with old data being overwritten until a stop command is received. Then stop capturing when memory is filled. This enables you to get some data before and some data after the stop pulse. Use the 'tr_en_cnt' register to determine where you are in your vector. 'Addr' register's MSb now indicates 'busy capturing'.
      |  3) Optionally capture a value on an input port to a register at the same time as the first data sample.
      |  4) Implement counters using DSP48Es to save resources.
      mask init: same as s_c107m32k_vlbi/snap_acc/ss
      settings: AttributesFormatString=|
      | 128 wide, 512 deep
      | debugID: 21079113
      mask TypeOptions storage: bram | dram
      mask Callback storage: snapshot_callback();
      mask TypeOptions dram_dimm: 1 | 2 | 3 | 4
      mask TypeOptions dram_clock: 200 | 250 | 266 | 300 | 333
      mask TypeOptions data_width: 8 | 16 | 32 | 64 | 128
  trig_delay : Subsystem  AncestorBlock=casper_library_delays/pipeline  mask(pipeline){csp_latency=2}
      mask prompts: csp_latency "Latency"
      mask help:
      | An explicitly laid-out delay line to avoid mapping to SRL16s
      | for use in pipelining to help achieve timing closure.
      mask init:
      | pipeline_init(gcb,'latency',csp_latency);
      settings: AttributesFormatString=Latency = %<latency>
      mask Display:
      | port_label('input', 1, 'd');
      | port_label('output', 1, 'q');
      | disp(['Z^-', num2str(csp_latency)]);
  we_delay : Subsystem  AncestorBlock=casper_library_delays/pipeline  mask(pipeline){csp_latency=2}
      mask prompts: csp_latency "Latency"
      mask help:
      | An explicitly laid-out delay line to avoid mapping to SRL16s
      | for use in pipelining to help achieve timing closure.
      mask init:
      | pipeline_init(gcb,'latency',csp_latency);
      settings: AttributesFormatString=Latency = %<latency>
      mask Display:
      | port_label('input', 1, 'd');
      | port_label('output', 1, 'q');
      | disp(['Z^-', num2str(csp_latency)]);
  arm_out : Outport
  wires:
  ss/1(arm_out) -> arm_out/1
  buscreate/1(bus_out) -> io_delay/1(d)
  io_delay/1(q) -> ss/1(din)
  in_sync0/1 -> assert_sync0/1
  assert_sync0/1 -> buscreate/1(in1)
  in_sync1/1 -> assert_sync1/1
  assert_sync1/1 -> buscreate/2(in2)
  in_data0/1 -> assert_data0/1
  assert_data0/1 -> buscreate/3(in3)
  in_data1/1 -> assert_data1/1
  assert_data1/1 -> buscreate/4(in4)
  in_rd_addr/1 -> assert_rd_addr/1
  assert_rd_addr/1 -> buscreate/5(in5)
  in_wr_addr/1 -> assert_wr_addr/1
  assert_wr_addr/1 -> buscreate/6(in6)
  in_valid/1 -> assert_valid/1
  assert_valid/1 -> buscreate/7(in7)
  in_tag/1 -> assert_tag/1
  assert_tag/1 -> buscreate/8(in8)
  we/1 -> we_delay/1(d)
  we_delay/1(q) -> ss/2(we)
  trig/1 -> trig_delay/1(d)
  trig_delay/1(q) -> ss/3(trig)

== system s_c107m32k_vlbi/cd_hmc/hmc_delay/status0 ==
  out_reord_jitter_err_cnt_pol0 : Inport
  out_reord_jitter_err_cnt_pol1 : Inport  Port=2
  out_hmc_err_cnt : Inport  Port=3
  assert_hmc_err_cnt : xbsIndex_r4/Assert  assert_type=on  type_source=Explicitly  gui_display_data_type=Fixed-point  arith_type=Unsigned  n_bits=10  bin_pt=0  preci_type=Single  exp_width=8  frac_width=24  assert_rate=off  rate_source=Explicitly  period=1  output_port=on  block_type=assert
  assert_reord_jitter_err_cnt_pol0 : xbsIndex_r4/Assert  assert_type=on  type_source=Explicitly  gui_display_data_type=Fixed-point  arith_type=Unsigned  n_bits=10  bin_pt=0  preci_type=Single  exp_width=8  frac_width=24  assert_rate=off  rate_source=Explicitly  period=1  output_port=on  block_type=assert
  assert_reord_jitter_err_cnt_pol1 : xbsIndex_r4/Assert  assert_type=on  type_source=Explicitly  gui_display_data_type=Fixed-point  arith_type=Unsigned  n_bits=10  bin_pt=0  preci_type=Single  exp_width=8  frac_width=24  assert_rate=off  rate_source=Explicitly  period=1  output_port=on  block_type=assert
  cast_gw : xbsIndex_r4/Convert  gui_display_data_type=Fixed-point  arith_type=Unsigned  n_bits=32  bin_pt=0  float_type=Single  exp_bits=8  fraction_bits=24  quantization=Truncate  overflow=Wrap  en=off  latency=1  pipeline=off  dbl_ovrd=off  block_type=convert
  concatenate : xbsIndex_r4/Concat  num_inputs=3  dbl_ovrd=off  block_type=concat
  io_delay : xbsIndex_r4/Delay  rst=off  infoeditControl=Selection of Reset will increase slice count due to use of real FFs and instead of SRLs  en=off  latency=0  reg_retiming=on  dbl_ovrd=off  block_type=delay
  reint1 : xbsIndex_r4/Reinterpret  force_arith_type=on  arith_type=Unsigned  force_bin_pt=on  bin_pt=0  block_type=reinterpret
  reint2 : xbsIndex_r4/Reinterpret  force_arith_type=on  arith_type=Unsigned  force_bin_pt=on  bin_pt=0  block_type=reinterpret
  reint3 : xbsIndex_r4/Reinterpret  force_arith_type=on  arith_type=Unsigned  force_bin_pt=on  bin_pt=0  block_type=reinterpret
  s_c107m32k_vlbi_cd_hmc_hmc_delay_status0_user_data_in : xbsIndex_r4/Gateway Out  inherit_from_input=off  hdl_port=on  rows=1  columns=1  UseAsDAC=off  DACChannel='1'  interface=None  automatic_assignment=on  address_offset=hex2dec('00')  intf_name=''  intf_description=''  timing_constraint=None  locs_specified=off  LOCs={}  io_standard={}  block_type=gatewayout
  sim_out : Terminator
  wires:
  concatenate/1 -> io_delay/1
  io_delay/1 -> cast_gw/1
  cast_gw/1 -> s_c107m32k_vlbi_cd_hmc_hmc_delay_status0_user_data_in/1
  s_c107m32k_vlbi_cd_hmc_hmc_delay_status0_user_data_in/1 -> sim_out/1
  out_reord_jitter_err_cnt_pol0/1 -> assert_reord_jitter_err_cnt_pol0/1
  assert_reord_jitter_err_cnt_pol0/1 -> reint1/1
  reint1/1 -> concatenate/1
  out_reord_jitter_err_cnt_pol1/1 -> assert_reord_jitter_err_cnt_pol1/1
  assert_reord_jitter_err_cnt_pol1/1 -> reint2/1
  reint2/1 -> concatenate/2
  out_hmc_err_cnt/1 -> assert_hmc_err_cnt/1
  assert_hmc_err_cnt/1 -> reint3/1
  reint3/1 -> concatenate/3
